simulink model "NREL5MW_FBNREL_SLOW1DOF"  (R2021b)
settings: Solver=ode4  StartTime=0.0  StopTime=Parameter.Time.TMax  FixedStep=Parameter.Time.dt  RelTol=1e-3  EnableMultiTasking=on
values from neighbouring files (symbols this model uses):
  Parameter = NREL5MWDefaultParameter_SLOW1DOF    [Exercise02_TorqueControllerDesign.m]    (also in Exercise02_TorqueControllerTest.m = NREL5MWDefaultParameter_FBNREL_TorqueController(Parameter))
settings Model: Creator=Phoenix_Shao  LastModifiedBy=david
settings SolverCC: AlgebraicLoopSolver=TrustRegion
settings DataIOCC: MaxDataPoints=1000000  SaveFormat=Array  DSMLogging=off  ReturnWorkspaceOutputs=off
settings OptimizationCC: ExpressionDepthLimit=2147483647  InitFltsAndDblsToZero=on  EfficientMapNaN2IntZero=off  LifeSpan=inf
settings DebuggingCC: SaveWithParameterizedLinksMsg=none  UnderspecifiedInitializationDetection=Classic  MergeDetectMultiDrivingBlocksExec=none  SignalResolutionControl=TryResolveAllWithWarning  SolverPrmCheckMsg=warning  MultiTaskDSMMsg=warning  MultiTaskCondExecSysMsg=none  FcnCallInpInsideContextMsg=warning  AllowSymbolicDim=off  StateNameClashWarn=warning  SFUnexpectedBacktrackingDiag=warning  SFNoUnconditionalDefaultTransitionDiag=warning  SFExecutionAtInitializationDiag=none  SFMachineParentedDataDiag=warning  ArithmeticOperatorsInVariantConditions=warning
settings HardwareCC: ProdBitPerPointer=32  ProdBitPerSizeT=32  ProdBitPerPtrDiffT=32  ProdLargestAtomicFloat=None  ProdIntDivRoundTo=Undefined  ProdEndianess=Unspecified  ProdWordSize=32  ProdHWDeviceType=32-bit Generic  TargetBitPerPointer=64  TargetBitPerSizeT=64  TargetBitPerPtrDiffT=64  TargetLongLongMode=on  TargetIntDivRoundTo=Zero  TargetEndianess=LittleEndian  TargetWordSize=64  TargetHWDeviceType=MATLAB Host  ProdEqTarget=off
settings ModelReferenceCC: PropagateSignalLabelsOutOfModel=off
settings SFSimCC: SimUseLocalCustomCode=off  SimParseCustomCode=off  CustomCodeUndefinedFunction=UseInterfaceOnly
settings RTWCC: SystemTargetFile=accel.tlc  TemplateMakefile=accel_default_tmf  RTWVerbose=off  RTWUseLocalCustomCode=off
settings CodeAppCC: MaxIdLength=128  StateflowObjectComments=on
settings STFCustomTargetCC: MATLABClassNameForMDSCustomization=Simulink.SoftwareTarget.TargetSpecificTriggerConfigurationBase  SystemTargetFile=accel.tlc
settings ConfigComp: CovMetricSettings=dw  CovSaveCumulativeToWorkspaceVar=on  CovSaveSingleToWorkspaceVar=on  CovExternalEMLEnable=off

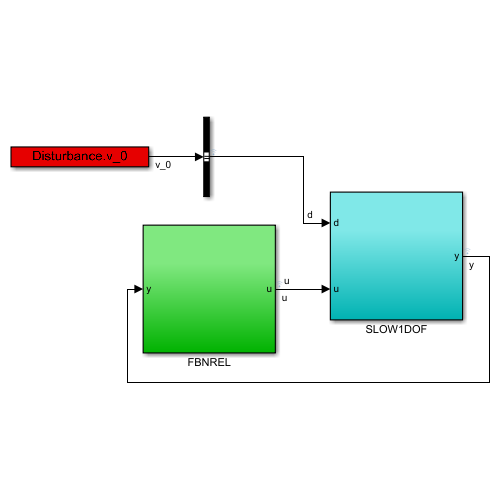
[thumbnail: Simulink's stored preview of the top-level diagram]
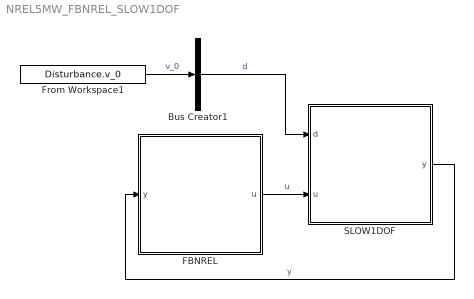
== system NREL5MW_FBNREL_SLOW1DOF ==
  Bus Creator1 : BusCreator  Inputs=1
  FBNREL : Subsystem
  From Workspace1 : FromWorkspace  VariableName=Disturbance.v_0
  SLOW1DOF : Subsystem
  wires:
  FBNREL/1(u) -> SLOW1DOF/2(u)  "u"
  Bus Creator1/1 -> SLOW1DOF/1(d)  "d"
  From Workspace1/1 -> Bus Creator1/1  "v_0"
  SLOW1DOF/1(y) -> FBNREL/1(y)  "y"

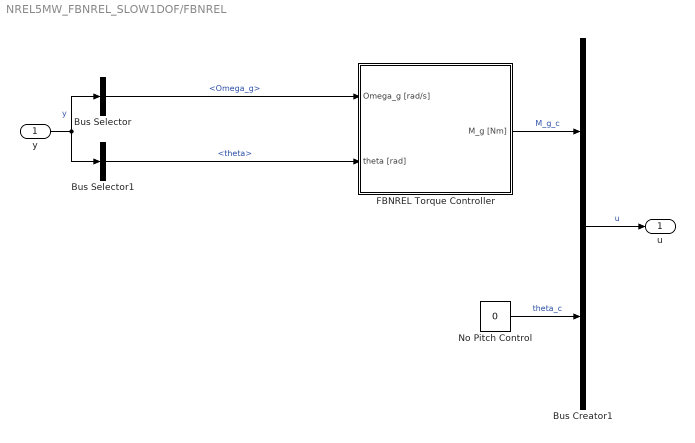
== system NREL5MW_FBNREL_SLOW1DOF/FBNREL ==
  y : Inport
  Bus Creator1 : BusCreator  Inputs=2
  Bus Selector : BusSelector  OutputSignals=Omega_g
  Bus Selector1 : BusSelector  OutputSignals=theta
  FBNREL Torque Controller : Subsystem
  No Pitch Control : Constant  Value=0
  u : Outport
  wires:
  Bus Selector1/1 -> FBNREL Torque Controller/2(theta [rad])  "<theta>"
  No Pitch Control/1 -> Bus Creator1/2  "theta_c"
  Bus Selector/1 -> FBNREL Torque Controller/1(Omega_g [rad/s])  "<Omega_g>"
  y/1 -> Bus Selector/1, Bus Selector1/1  "y"
  FBNREL Torque Controller/1(M_g [Nm]) -> Bus Creator1/1  "M_g_c"
  Bus Creator1/1 -> u/1  "u"

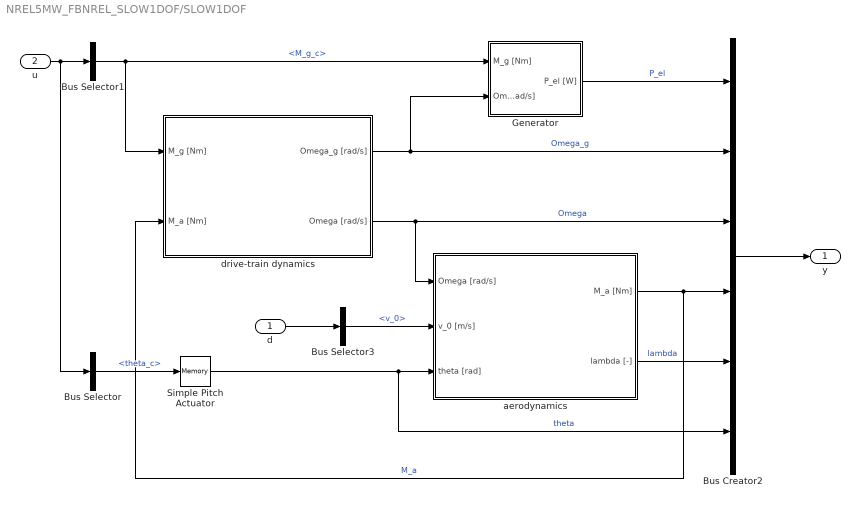
== system NREL5MW_FBNREL_SLOW1DOF/SLOW1DOF ==
  d : Inport
  u : Inport  Port=2
  Bus Creator2 : BusCreator  Inputs=6
  Bus Selector : BusSelector  OutputSignals=theta_c
  Bus Selector1 : BusSelector  OutputSignals=M_g_c
  Bus Selector3 : BusSelector  OutputSignals=v_0
  Generator : Subsystem
  Simple Pitch Actuator : Memory  InitialCondition=Parameter.IC.theta
  aerodynamics : Subsystem
  drive-train dynamics : Subsystem
  y : Outport
  wires:
  Bus Selector3/1 -> aerodynamics/2(v_0 [m/s])  "<v_0>"
  d/1 -> Bus Selector3/1
  aerodynamics/2(lambda [-]) -> Bus Creator2/5  "lambda"
  Bus Selector/1 -> Simple Pitch Actuator/1  "<theta_c>"
  u/1 -> Bus Selector/1, Bus Selector1/1
  Bus Creator2/1 -> y/1
  aerodynamics/1(M_a [Nm]) -> Bus Creator2/4, drive-train dynamics/2(M_a [Nm])  "M_a"
  drive-train dynamics/2(Omega [rad/s]) -> Bus Creator2/3, aerodynamics/1(Omega [rad/s])  "Omega"
  drive-train dynamics/1(Omega_g [rad/s]) -> Bus Creator2/2, Generator/2(Omega_g [rad/s])  "Omega_g"
  Generator/1(P_el [W]) -> Bus Creator2/1  "P_el"
  Bus Selector1/1 -> drive-train dynamics/1(M_g [Nm]), Generator/1(M_g [Nm])  "<M_g_c>"
  Simple Pitch Actuator/1 -> Bus Creator2/6, aerodynamics/3(theta [rad])  "theta"

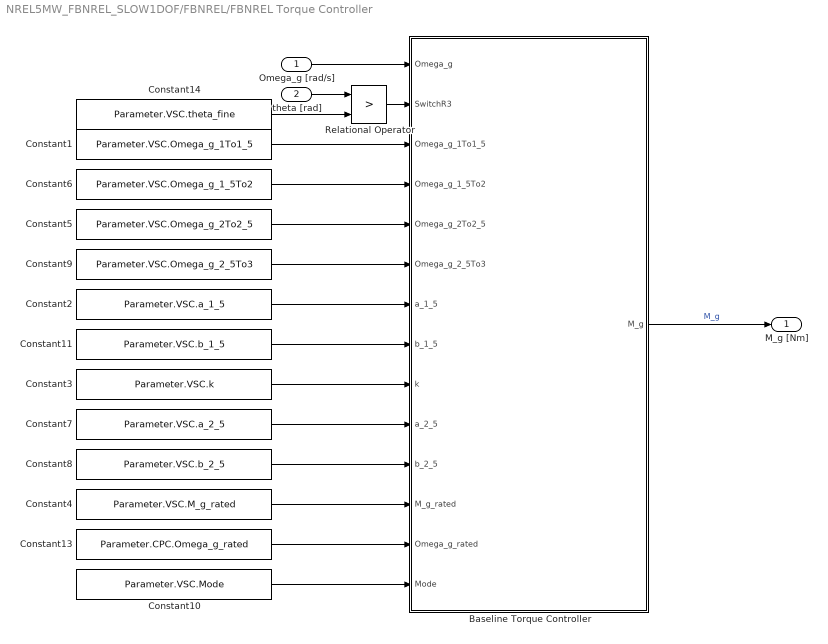
== system NREL5MW_FBNREL_SLOW1DOF/FBNREL/FBNREL Torque Controller ==
  Omega_g [rad/s] : Inport
  theta [rad] : Inport  Port=2
  Baseline Torque Controller : MATLAB Function  TreatAsAtomicUnit=on
  Constant1 : Constant  Value=Parameter.VSC.Omega_g_1To1_5
  Constant10 : Constant  Value=Parameter.VSC.Mode
  Constant11 : Constant  Value=Parameter.VSC.b_1_5
  Constant13 : Constant  Value=Parameter.CPC.Omega_g_rated
  Constant14 : Constant  Value=Parameter.VSC.theta_fine
  Constant2 : Constant  Value=Parameter.VSC.a_1_5
  Constant3 : Constant  Value=Parameter.VSC.k
  Constant4 : Constant  Value=Parameter.VSC.M_g_rated
  Constant5 : Constant  Value=Parameter.VSC.Omega_g_2To2_5
  Constant6 : Constant  Value=Parameter.VSC.Omega_g_1_5To2
  Constant7 : Constant  Value=Parameter.VSC.a_2_5
  Constant8 : Constant  Value=Parameter.VSC.b_2_5
  Constant9 : Constant  Value=Parameter.VSC.Omega_g_2_5To3
  Relational Operator : RelationalOperator  Operator=>  OutDataTypeStr=boolean  RndMeth=Nearest
  M_g [Nm] : Outport
  wires:
  Constant13/1 -> Baseline Torque Controller/13(Omega_g_rated)
  Constant11/1 -> Baseline Torque Controller/8(b_1_5)
  Constant2/1 -> Baseline Torque Controller/7(a_1_5)
  Constant10/1 -> Baseline Torque Controller/14(Mode)
  Constant3/1 -> Baseline Torque Controller/9(k)
  Constant7/1 -> Baseline Torque Controller/10(a_2_5)
  Constant8/1 -> Baseline Torque Controller/11(b_2_5)
  Constant4/1 -> Baseline Torque Controller/12(M_g_rated)
  Constant9/1 -> Baseline Torque Controller/6(Omega_g_2_5To3)
  Constant6/1 -> Baseline Torque Controller/4(Omega_g_1_5To2)
  Constant5/1 -> Baseline Torque Controller/5(Omega_g_2To2_5)
  Constant1/1 -> Baseline Torque Controller/3(Omega_g_1To1_5)
  Baseline Torque Controller/1(M_g) -> M_g [Nm]/1  "M_g"
  Omega_g [rad/s]/1 -> Baseline Torque Controller/1(Omega_g)
  Constant14/1 -> Relational Operator/2
  theta [rad]/1 -> Relational Operator/1
  Relational Operator/1 -> Baseline Torque Controller/2(SwitchR3)

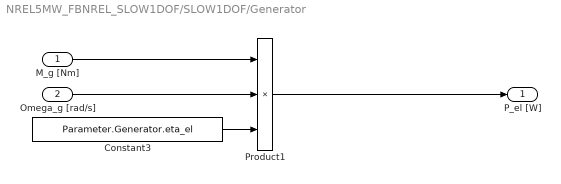
== system NREL5MW_FBNREL_SLOW1DOF/SLOW1DOF/Generator ==
  M_g [Nm] : Inport
  Omega_g [rad/s] : Inport  Port=2
  Constant3 : Constant  Value=Parameter.Generator.eta_el
  Product1 : Product  Inputs=***  RndMeth=Zero
  P_el [W] : Outport
  wires:
  Constant3/1 -> Product1/3
  M_g [Nm]/1 -> Product1/1
  Omega_g [rad/s]/1 -> Product1/2
  Product1/1 -> P_el [W]/1

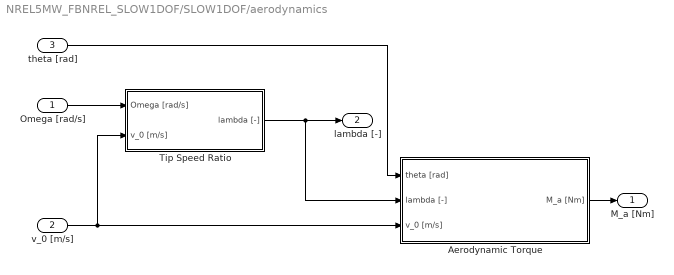
== system NREL5MW_FBNREL_SLOW1DOF/SLOW1DOF/aerodynamics ==
  Omega [rad/s] : Inport
  v_0 [m/s] : Inport  Port=2
  theta [rad] : Inport  Port=3
  Aerodynamic Torque : Subsystem
  Tip Speed Ratio : Subsystem
  M_a [Nm] : Outport
  lambda [-] : Outport  Port=2
  wires:
  Tip Speed Ratio/1(lambda [-]) -> lambda [-]/1, Aerodynamic Torque/2(lambda [-])
  v_0 [m/s]/1 -> Aerodynamic Torque/3(v_0 [m/s]), Tip Speed Ratio/2(v_0 [m/s])
  Omega [rad/s]/1 -> Tip Speed Ratio/1(Omega [rad/s])
  Aerodynamic Torque/1(M_a [Nm]) -> M_a [Nm]/1
  theta [rad]/1 -> Aerodynamic Torque/1(theta [rad])

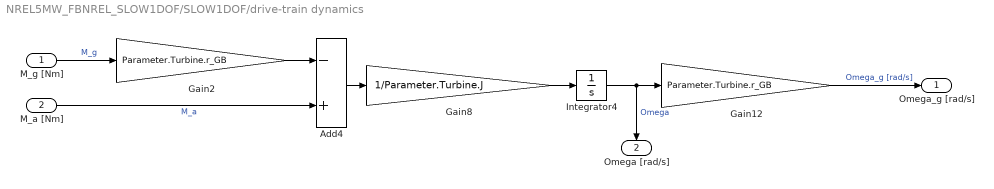
== system NREL5MW_FBNREL_SLOW1DOF/SLOW1DOF/drive-train dynamics ==
  M_g [Nm] : Inport
  M_a [Nm] : Inport  Port=2
  Add4 : Sum  Inputs=-+
  Gain12 : Gain  Gain=Parameter.Turbine.r_GB  SaturateOnIntegerOverflow=on  OutDataTypeStr=Inherit: Same as input  ParamDataTypeStr=Inherit: Same as input
  Gain2 : Gain  Gain=Parameter.Turbine.r_GB  SaturateOnIntegerOverflow=on  OutDataTypeStr=Inherit: Same as input  ParamDataTypeStr=Inherit: Same as input
  Gain8 : Gain  Gain=1/Parameter.Turbine.J  SaturateOnIntegerOverflow=on  OutDataTypeStr=Inherit: Same as input  ParamDataTypeStr=Inherit: Same as input
  Integrator4 : Integrator  InitialCondition=Parameter.IC.Omega
  Omega_g [rad/s] : Outport
  Omega [rad/s] : Outport  Port=2
  wires:
  M_a [Nm]/1 -> Add4/2  "M_a"
  Integrator4/1 -> Omega [rad/s]/1, Gain12/1  "Omega"
  Add4/1 -> Gain8/1
  Gain8/1 -> Integrator4/1
  Gain2/1 -> Add4/1
  Gain12/1 -> Omega_g [rad/s]/1  "Omega_g [rad/s]"
  M_g [Nm]/1 -> Gain2/1  "M_g"

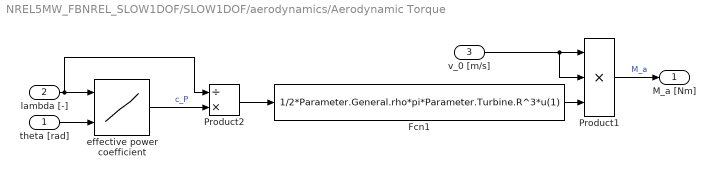
== system NREL5MW_FBNREL_SLOW1DOF/SLOW1DOF/aerodynamics/Aerodynamic Torque ==
  theta [rad] : Inport
  lambda [-] : Inport  Port=2
  v_0 [m/s] : Inport  Port=3
  Fcn1 : Fcn  Expr=1/2*Parameter.General.rho*pi*Parameter.Turbine.R^3*u(1)
  Product1 : Product  Inputs=3  RndMeth=Zero
  Product2 : Product  Inputs=/*  RndMeth=Zero
  effective power coefficient : Lookup2D  RowIndex=Parameter.Turbine.SS.lambda  ColumnIndex=Parameter.Turbine.SS.theta  Table=Parameter.Turbine.SS.c_P
  M_a [Nm] : Outport
  wires:
  Product2/1 -> Fcn1/1
  effective power coefficient/1 -> Product2/2  "c_P"
  v_0 [m/s]/1 -> Product1/2, Product1/1
  theta [rad]/1 -> effective power coefficient/2
  lambda [-]/1 -> Product2/1, effective power coefficient/1
  Fcn1/1 -> Product1/3
  Product1/1 -> M_a [Nm]/1  "M_a"

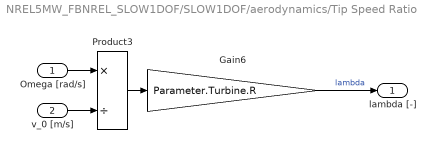
== system NREL5MW_FBNREL_SLOW1DOF/SLOW1DOF/aerodynamics/Tip Speed Ratio ==
  Omega [rad/s] : Inport
  v_0 [m/s] : Inport  Port=2
  Gain6 : Gain  Gain=Parameter.Turbine.R  SaturateOnIntegerOverflow=on  OutDataTypeStr=Inherit: Same as input  ParamDataTypeStr=Inherit: Same as input
  Product3 : Product  Inputs=*/  RndMeth=Zero
  lambda [-] : Outport
  wires:
  Gain6/1 -> lambda [-]/1  "lambda"
  v_0 [m/s]/1 -> Product3/2
  Omega [rad/s]/1 -> Product3/1
  Product3/1 -> Gain6/1

== matlab function NREL5MW_FBNREL_SLOW1DOF/FBNREL/FBNREL Torque Controller/Baseline Torque Controller ==
  settings: fimath=|
      | fimath(...
      | 'RoundMode', 'floor',...
      | 'OverflowMode', 'wrap',...
      | 'ProductMode', 'KeepLSB', 'ProductWordLength', 32,...
      | 'SumMode', 'KeepLSB', 'SumWordLength', 32,...
      | 'CastBeforeSum', false)
  data: Omega_g input; SwitchR3 input; Omega_g_1To1_5 input; Omega_g_1_5To2 input; Omega_g_2To2_5 input; Omega_g_2_5To3 input; a_1_5 input; b_1_5 input; k input; a_2_5 input; b_2_5 input; M_g output; M_g_rated input; Omega_g_rated input; Mode input
function M_g = BaselineVSControl(Omega_g,SwitchR3,...  	% signals
    Omega_g_1To1_5,Omega_g_1_5To2,...
    Omega_g_2To2_5,Omega_g_2_5To3,...                   % region limits
    a_1_5,b_1_5,...                                    	% Region 1.5 parameters
    k,...                                             	% Region   2 parameters
    a_2_5,b_2_5,...                                    	% Region 2.5 parameters
    M_g_rated,Omega_g_rated,Mode)                       % Region   3 parameters

M_g = 0;    % Dummy

end
